simulink model "state_estimator"  (R2025b)
settings: Solver=VariableStepAuto  StartTime=0.0  StopTime=10  RelTol=1e-3
InitFcn:
  | %% State Estimator
  | p_init  = [0,0,0];
  | v_init  = [0,0,0];
  | q_init  = [1,0,0,0];
  | bg_init = [1.045715,0.002947,-0.517855];
  | ba_high_init = [-7.395250,-4.820243,-18.177021];
  | ba_low_init = [-0.021725, 0.062643, -0.022747];
  | 
  | taug_init = [1.105; 1.105; 1.105];
  | taua_high_init = [8.731; 8.731; 8.731];
  | qg_init = [4.390573e-05; 2.319960e-05; 1.494807e-05];
  | qa_high_init = [8.774166e-04; 7.720775e-04; 1.336849e-03];
  | 
  | x_init = [p_init, v_init, q_init, bg_init, ba_high_init, ba_low_init]';
  | P_init = zeros(19);
  | dt = 1/1000;
  | %% Sensors
  | % Low-g accelerometer
  | dt_lowaccel = 1/120;
  | ba_low_init = [-0.021725; 0.062643; -0.022747];
  | taua_low = [1.437; 1.437; 1.437];
  | qa_low = [1.483796e-6; 1.224280e-6; 1.983171e-6];
  | noise_std_lowaccel = [0.020005; 0.021677; 0.025995];
  | quant_step_lowaccel = 0.004905;
  | 
  | % Gyro
  | dt_gyro = 1/120;
  | gyro_bias_init = [1.045715; 0.002947; -0.517855];
  | gyro_tau = [1.105; 1.105; 1.105];
  | gyro_drift_variance = [4.390573e-5; 2.319960e-5; 1.494807e-5];
  | gyro_noise_std = [0.130937; 0.093580; 0.075444];
  | gyro_quant_step = 0.05;
  | 
  | % High-g acceleromter
  | dt_highaccel = 1/120;
  | highaccel_bias_init = [-7.395250; -4.820243; -18.177021];
  | highaccel_tau = [8.731; 8.731; 8.731];
  | highaccel_drift_variance = [8.774166e-4; 7.720775e-4; 1.336849e-3];
  | highaccel_noise_std = [1.645664; 1.487596; 1.836378];
  | highaccel_quant_step = 0.5;
  | 
  | % Barometer [K Pa]
  | dt_baro = 1/50;
  | baro_bias_init = [0; 0];
  | baro_tau = [11.9906; 88.5141];
  | baro_drift_variance = [4.1889e-8; 2.9560e-4];
  | baro_noise_std = [0.01; 0.35];
  | baro_quant_step = [0.01; 0.06];
  | 
  | % Magnetometer
  | dt_mag = 1/50;
  | mag_bias_init = [0; 0; 0];
  | mag_tau = [6.9630; 7.8914; 6.3777];
  | mag_drift_variance = [1.1384e-11; 2.9369e-11; 4.0735e-11];
  | mag_noise_std = [1.2; 1.2; 1.2];
  | mag_quant_step = [0.0625; 0.0625; 0.0625];
  | 
  | % GPS
  | dt_gps = 1/50;
  | gps_bias_init = [0; 0; 0; 0; 0; 0; 0; 0; 0];
  | gps_tau = [116.2031; 204.0083; 88.1618; 0.3353; 1.4466; 0.8506; inf; inf; inf];
  | gps_drift_variance = [6.1178e-20; 7.8958e-20; 1.0101e-2; 1.1742e-4; 6.3880e-5; 9.5787e-5; 0; 0; 0];
  | gps_noise_std = [1.35e-7; 1.35e-7; 1.35e-8; 5e-5; 5e-5; 5e-5; 0; 0; 0];
  | gps_quant_step = [0.5e-7; 0.5e-7; 5e-4; 5e-4; 5e-4; 5e-4; 1; 1; 0.1];
  | 
  | % LiDAR
  | dt_lidar = 1/50;
  | lidar_bias_init = 0.01;
  | lidar_tau = 120;
  | lidar_drift_variance = 1e-6;
  | lidar_noise_std = 0.03;
  | lidar_quant_step = 0.01;
  | lidar_min_range = 0.2;
  | lidar_max_range = 8.0;
undefined symbols (not defined in the file): DiscIntNeverNeededParam
settings Model: LastModifiedBy=Admin

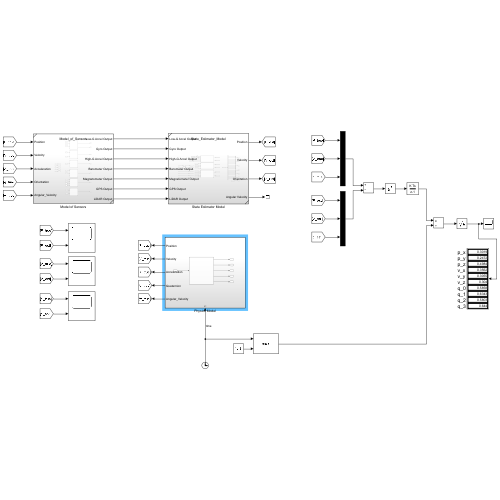
[thumbnail: Simulink's stored preview of the top-level diagram]
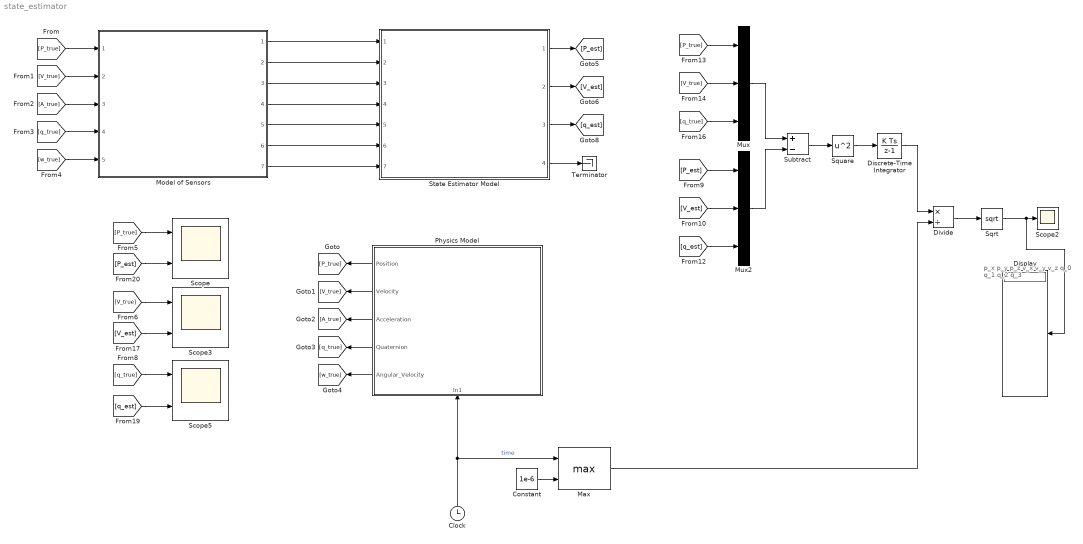
== system state_estimator ==
  note: p_x
      | p_y
      | p_z
      | v_x
      | v_y
      | v_z
      | q_0
      | q_1
      | q_2
      | q_3
  Clock : Clock
  Constant : Constant  Value=1e-6
  Discrete-Time Integrator : DiscreteIntegrator  SampleTime=-1  ICPrevOutput=DiscIntNeverNeededParam  ICPrevScaledInput=DiscIntNeverNeededParam
  Display : Display
  Divide : Product  Inputs=*/
  Max : MinMax  Function=max  Inputs=2
  Model of Sensors : Subsystem  ReferencedSubsystem=Model_of_Sensors
  Mux : Mux  Inputs=3
  Mux2 : Mux  Inputs=3
  Physics Model : Subsystem
      settings: PortSchema="{\"entries\":[{\"content\":{\"sides\":[{\"content\":{\"connectorIds\":[\"Out1\",\"Out2\",\"Out3\",\"Out4\",\"Out5\"]},\"type\":\"ConnectorPlacement.EquallySpacedRectSide\",\"uuid\":\"d973089c-7b51-4721-858e-49b2da9ba2e2\"},{\"content\":{\"side\":\"RIGHT\"},\"type\":\"ConnectorPlacement.EquallySpacedRectSide\",\"uuid\":\"a0a62891-f020-44a5-9f44-1534f6d7597c\"},{\"content\":{\"side\":\"TOP\"},\"type\":\"ConnectorPlacement.EquallySpacedRectSide\",\"uuid\":\"420ffd3e-2259-443b-b734-66425db33e5d\"},{\"content\":{\"connectorIds\":[\"In1\"],\"side\":\"BOTTOM\"},\"type\":\"ConnectorPlacement.EquallySpacedRectSide\",\"uuid\":\"61b4c197-8443-47ca-8602-966eda63e0fb\"}]},\"type\":\"ConnectorPlacement.EquallySpacedConnector\",\"uuid\":\"7be80f26-ca88-418d-b859-dfd10cd1bf87\"}],\"packageUris\":[\"http://schema.mathworks.com/mf0/Connector/R2020b\"],\"version\":\"1.0\"}"
  Scope : Scope  NumInputPorts=2
      settings: ActiveDisplayYMinimum=-2.5463099724280132  ActiveDisplayYMaximum=2.9167897518521206  DataLoggingVariableName=ScopeData3
  Scope2 : Scope
      settings: ActiveDisplayYMinimum=-1  ActiveDisplayYMaximum=1  DataLoggingVariableName=ScopeData2
  Scope3 : Scope  NumInputPorts=2
      settings: ActiveDisplayYMinimum=-1  ActiveDisplayYMaximum=1  DataLoggingVariableName=ScopeData7
  Scope5 : Scope  NumInputPorts=2
      settings: ActiveDisplayYMinimum=-0.929971224193129  ActiveDisplayYMaximum=1.2144412436130687  DataLoggingVariableName=ScopeData6
  Sqrt : Sqrt
  Square : Math  Operator=square
  State Estimator Model : Subsystem  ReferencedSubsystem=State_Estimator_Model
  Subtract : Sum  Inputs=+-
  Terminator : Terminator
  wires:
  Clock/1 -> Max/1, Physics Model/1(In1)  "time"
  Model of Sensors/1 -> State Estimator Model/1
  Model of Sensors/3 -> State Estimator Model/3
  Model of Sensors/4 -> State Estimator Model/4
  Model of Sensors/5 -> State Estimator Model/5
  Model of Sensors/6 -> State Estimator Model/6
  Model of Sensors/2 -> State Estimator Model/2
  Subtract/1 -> Square/1
  Discrete-Time Integrator/1 -> Divide/1
  Square/1 -> Discrete-Time Integrator/1
  Divide/1 -> Sqrt/1
  Constant/1 -> Max/2
  Physics Model/1(Position) -> [P_true]
  [P_true] -> Model of Sensors/1
  Physics Model/2(Velocity) -> [V_true]
  Physics Model/3(Acceleration) -> [A_true]
  Physics Model/4(Quaternion) -> [q_true]
  [V_true] -> Model of Sensors/2
  [A_true] -> Model of Sensors/3
  [q_true] -> Model of Sensors/4
  [w_true] -> Model of Sensors/5
  Physics Model/5(Angular_Velocity) -> [w_true]
  [V_true] -> Scope3/1
  [q_true] -> Scope5/1
  [P_true] -> Scope/1
  State Estimator Model/1 -> [P_est]
  State Estimator Model/2 -> [V_est]
  State Estimator Model/3 -> [q_est]
  [q_true] -> Mux/3
  [V_true] -> Mux/2
  [P_true] -> Mux/1
  [P_est] -> Mux2/1
  [V_est] -> Mux2/2
  [q_est] -> Mux2/3
  [P_est] -> Scope/2
  [V_est] -> Scope3/2
  [q_est] -> Scope5/2
  Mux/1 -> Subtract/1
  Mux2/1 -> Subtract/2
  Max/1 -> Divide/2
  Sqrt/1 -> Display/1, Scope2/1
  Model of Sensors/7 -> State Estimator Model/7
  State Estimator Model/4 -> Terminator/1

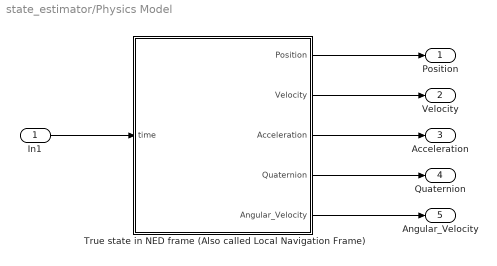
== system state_estimator/Physics Model ==
  In1 : Inport
  True state in NED frame (Also called Local Navigation Frame) : MATLAB Function  TreatAsAtomicUnit=on
  Position : Outport
  Velocity : Outport  Port=2
  Acceleration : Outport  Port=3
  Quaternion : Outport  Port=4
  Angular_Velocity : Outport  Port=5
  wires:
  In1/1 -> True state in NED frame (Also called Local Navigation Frame)/1(time)
  True state in NED frame (Also called Local Navigation Frame)/4(Quaternion) -> Quaternion/1
  True state in NED frame (Also called Local Navigation Frame)/2(Velocity) -> Velocity/1
  True state in NED frame (Also called Local Navigation Frame)/1(Position) -> Position/1
  True state in NED frame (Also called Local Navigation Frame)/3(Acceleration) -> Acceleration/1
  True state in NED frame (Also called Local Navigation Frame)/5(Angular_Velocity) -> Angular_Velocity/1

== matlab function state_estimator/Physics Model/True state in NED frame (Also called Local Navigation Frame) ==
  data: time input; Position output; Velocity output; Acceleration output; Quaternion output; Angular_Velocity output
function [Position, Velocity, Acceleration, Quaternion, Angular_Velocity] = fcn(time)
% Frames:
% - Position, Velocity, Acceleration in NED
% - Quaternion scalar-first [q0; q1; q2; q3]
% - Angular_Velocity = [p; q; r] in rad/s

% -----------------------------
% Trajectory configuration
% -----------------------------
T.x0       = 0.0;   T.xi = 2.0;   T.xf = 0.0;
T.y0       = 0.0;   T.yi = 2.0;   T.yf = 0.0;
T.z0       = 0.0;   T.zi = -2.0;   T.zf = 0.0;
T.t1       = 5.0;
T.t2       = 5.0;
T.dt_blend = 2.0;
T.frac_tb  = 0.20;
T.useStep  = false;

% -----------------------------
% Translational motion
% -----------------------------
[Position, Velocity, Acceleration] = trapezoidalRefBlockXYZ(time, T);

% Position     = [0; 0; -5];
% Velocity     = [0; 0; 0];
% Acceleration = [0; 0; 0];
% -----------------------------
% Position trajectory in NED
% Hover at 5 m, then climb/descent sinusoid
% Ground plane is D = 0
% Above ground means D is negative
% -----------------------------
% h0 = 5;              % mean height above ground [m]
% Ah = 2;              % height oscillation amplitude [m]
% fh = 0.05;           % height frequency [Hz]
% 
% h = h0 + Ah*sin(2*pi*fh*time);
% 
% hdot = Ah*2*pi*fh*cos(2*pi*fh*time);
% hddot = -Ah*(2*pi*fh)^2*sin(2*pi*fh*time);
% 
% Position = [0; 0; -h];
% Velocity = [0; 0; -hdot];
% Acceleration = [0; 0; -hddot];

% -----------------------------
% Rotational motion
% Constant roll rate + constant yaw rate
% This exercises:
%   - accel update (roll/pitch correction)
%   - mag update   (yaw correction)
%   - gyro update  (rate correction)
% -----------------------------
roll_amp  = deg2rad(0);
pitch_amp = deg2rad(0);
yaw_amp   = deg2rad(0);

wr = 0.5;
wp = 0.3;
wy = 0.2;

roll  = roll_amp  * sin(wr*time);
pitch = pi/2 + pitch_amp*sin(wp*time);
yaw   = yaw_amp   * sin(wy*time);

roll_dot  = roll_amp  * wr * cos(wr*time);
pitch_dot = pitch_amp * wp * cos(wp*time);
yaw_dot   = yaw_amp   * wy * cos(wy*time);

p = roll_dot - yaw_dot*sin(pitch);
q = pitch_dot*cos(roll) + yaw_dot*sin(roll)*cos(pitch);
r = -pitch_dot*sin(roll) + yaw_dot*cos(roll)*cos(pitch);

Angular_Velocity = [p; q; r];

% -----------------------------
% Quaternion from Euler ZYX
% -----------------------------
cr = cos(roll/2);  sr = sin(roll/2);
cp = cos(pitch/2); sp = sin(pitch/2);
cy = cos(yaw/2);   sy = sin(yaw/2);

Quaternion = [cr*cp*cy + sr*sp*sy;
              sr*cp*cy - cr*sp*sy;
              cr*sp*cy + sr*cp*sy;
              cr*cp*sy - sr*sp*cy];
end
